simulink model "mpct_simple"  (R2025b)
settings: Solver=FixedStepDiscrete  StartTime=0  StopTime=240  FixedStep=1  RelTol=1e-3
PostLoadFcn:
  | addpath(fileparts(get_param(bdroot,'FileName')));
InitFcn:
  | addpath(fileparts(get_param(bdroot,'FileName'))); clear simple_mpct_step simple_rg_step;
model workspace (MAT data in the model file):
  reference_data.time = [0; 10; 80; 160; 240]
  reference_data.signals.values = [0; 0.7; 1.2; 0.3; 0.3]
  reference_data.signals.dimensions = 1
settings Model: Creator=alosw  LastModifiedBy=alosw
settings DataIOCC: SaveOutput=off  SignalLogging=off

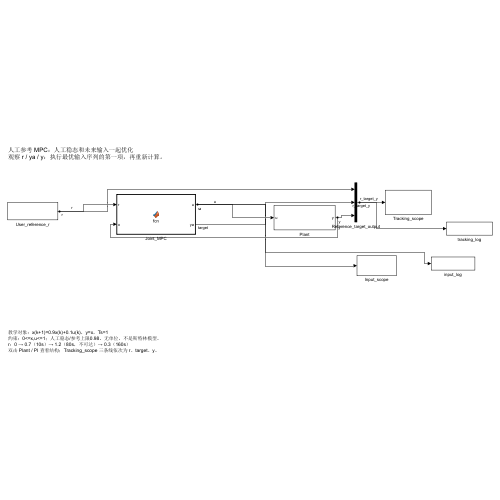
[thumbnail: Simulink's stored preview of the top-level diagram]
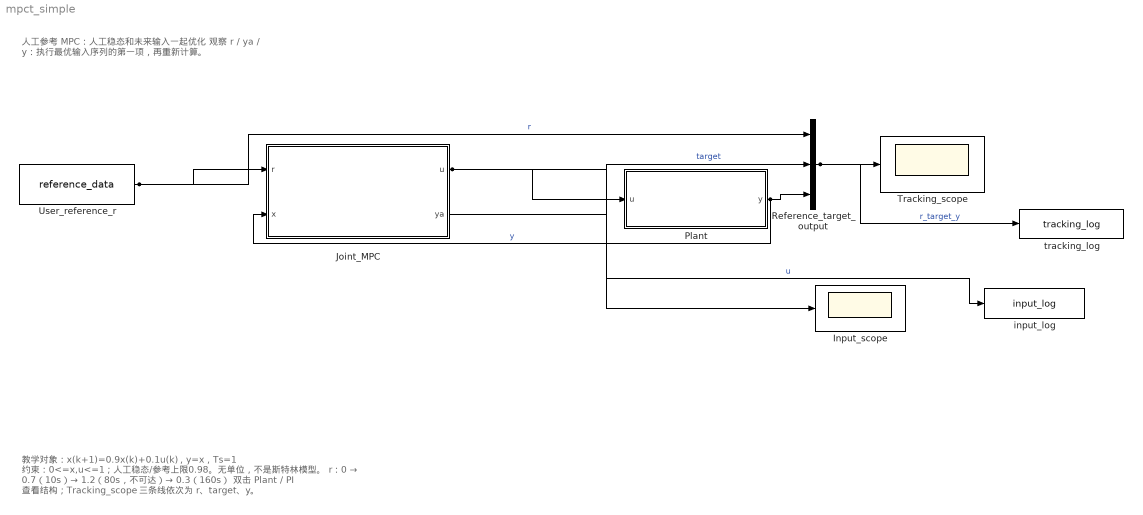
== system mpct_simple ==
  note: 人工参考 MPC：人工稳态和未来输入一起优化
      | 观察 r / ya / y：执行最优输入序列的第一项，再重新计算。
  note: 教学对象：x(k+1)=0.9x(k)+0.1u(k)，y=x，Ts=1
      | 约束：0<=x,u<=1；人工稳态/参考上限0.98。无单位，不是斯特林模型。
      | r：0 → 0.7（10s）→ 1.2（80s，不可达）→ 0.3（160s）
      | 双击 Plant / PI 查看结构；Tracking_scope 三条线依次为 r、target、y。
  Input_scope : Scope
  Joint_MPC : MATLAB Function  TreatAsAtomicUnit=on
  Plant : Subsystem
  Reference_target_output : Mux  Inputs=3
  Tracking_scope : Scope
  User_reference_r : FromWorkspace  VariableName=reference_data  SampleTime=1  Interpolate=off  OutputAfterFinalValue=Holding final value
  input_log : ToWorkspace  VariableName=input_log  SampleTime=-1
  tracking_log : ToWorkspace  VariableName=tracking_log  SampleTime=-1
  wires:
  User_reference_r/1 -> Joint_MPC/1(r), Reference_target_output/1  "r"
  Plant/1(y) -> Joint_MPC/2(x), Reference_target_output/3  "y"
  Joint_MPC/1(u) -> Plant/1(u), Input_scope/1, input_log/1  "u"
  Joint_MPC/2(ya) -> Reference_target_output/2  "target"
  Reference_target_output/1 -> Tracking_scope/1, tracking_log/1  "r_target_y"

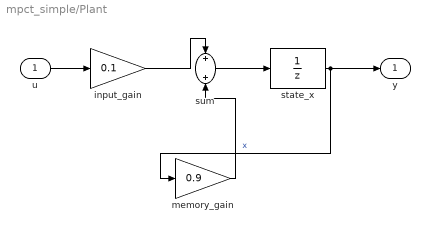
== system mpct_simple/Plant ==
  u : Inport
  input_gain : Gain  Gain=0.1
  memory_gain : Gain  Gain=0.9
  state_x : UnitDelay  HasFrameUpgradeWarning=on
  sum : Sum
  y : Outport
  wires:
  u/1 -> input_gain/1
  input_gain/1 -> sum/1
  sum/1 -> state_x/1
  state_x/1 -> y/1, memory_gain/1  "x"
  memory_gain/1 -> sum/2

== matlab function mpct_simple/Joint_MPC ==
  data: r input; u output; x input; ya output
function [u,ya] = fcn(r,x)
% Joint optimization of artificial equilibrium and future inputs.
coder.extrinsic('simple_mpct_step');
a=zeros(2,1);
a=simple_mpct_step([r;x]);
u=a(1);
ya=a(2);
end
